simulink model "System_D_passive_simscape"  (R2026a)
settings: Solver=ode23t  StopTime=0.02
libraries: fl_lib x25, nesl_utility x5
settings Model: Creator=mads  LastModifiedBy=mads

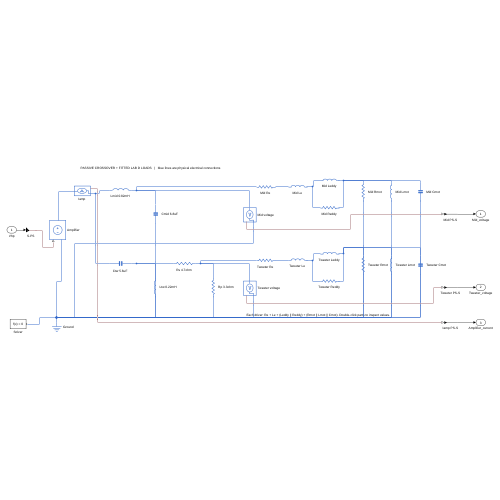
[thumbnail: Simulink's stored preview of the top-level diagram]
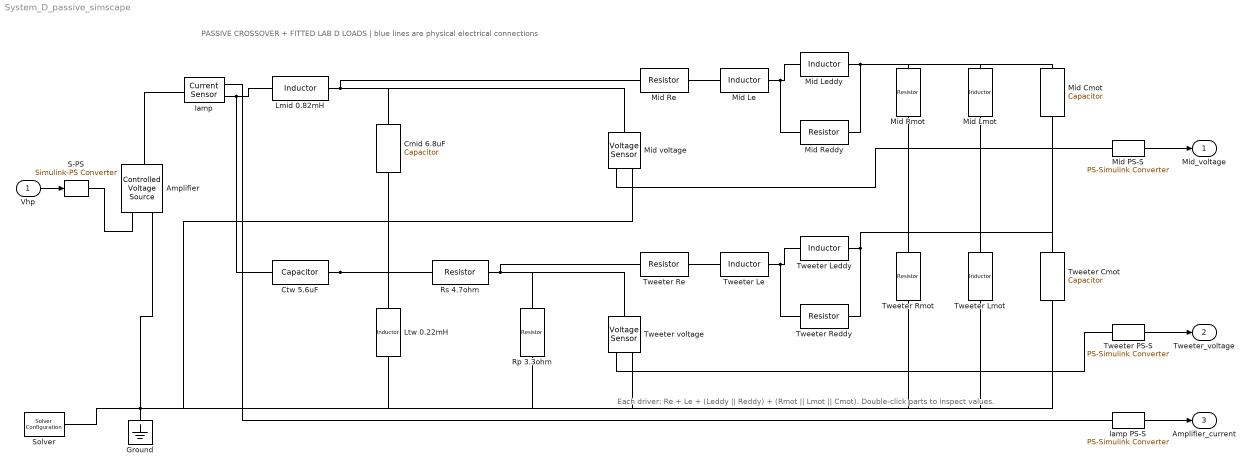
== system System_D_passive_simscape ==
  note: PASSIVE CROSSOVER + FITTED LAB D LOADS | blue lines are physical electrical connections
  note: Each driver: Re + Le + (Leddy || Reddy) + (Rmot || Lmot || Cmot). Double-click parts to inspect values.
  Vhp : Inport
  Amplifier : fl_lib/Electrical/Electrical Sources/Controlled Voltage Source
  Cmid 6.8uF : fl_lib/Electrical/Electrical Elements/Capacitor  c=6.8e-06 F  r=0 Ohm  g=0 1/Ohm  i_specify=off  i_priority=None  i=0 A  i_nominal_specify=off  i_nominal_value=1  i_nominal_unit=A  v_specify=off  v_priority=None  v=0 V  v_nominal_specify=off  v_nominal_value=1  v_nominal_unit=V  vc_specify=off  vc_priority=High  vc=0 V  vc_nominal_specify=off  vc_nominal_value=1  vc_nominal_unit=V
  Ctw 5.6uF : fl_lib/Electrical/Electrical Elements/Capacitor  c=5.6e-06 F  r=0 Ohm  g=0 1/Ohm  i_specify=off  i_priority=None  i=0 A  i_nominal_specify=off  i_nominal_value=1  i_nominal_unit=A  v_specify=off  v_priority=None  v=0 V  v_nominal_specify=off  v_nominal_value=1  v_nominal_unit=V  vc_specify=off  vc_priority=High  vc=0 V  vc_nominal_specify=off  vc_nominal_value=1  vc_nominal_unit=V
  Ground : fl_lib/Electrical/Electrical Elements/Electrical Reference
  Iamp : fl_lib/Electrical/Electrical Sensors/Current Sensor
  Iamp PS-S : nesl_utility/PS-Simulink Converter  PhysicalDomain=network_engine_domain  SubClassName=ps_output  LeftPortType=input  RightPortType=output  PseudoPeriodic=off  Frequencies=[]  VectorFormat=inherit  Unit=A  AffineConversion=off
  Lmid 0.82mH : fl_lib/Electrical/Electrical Elements/Inductor  l=0.00082 H  r=0 Ohm  g=0 1/Ohm  i_specify=off  i_priority=None  i=0 A  i_nominal_specify=off  i_nominal_value=1  i_nominal_unit=A  v_specify=off  v_priority=None  v=0 V  v_nominal_specify=off  v_nominal_value=1  v_nominal_unit=V  i_L_specify=off  i_L_priority=High  i_L=0 A  i_L_nominal_specify=off  i_L_nominal_value=1  i_L_nominal_unit=A
  Ltw 0.22mH : fl_lib/Electrical/Electrical Elements/Inductor  l=0.00022 H  r=0 Ohm  g=0 1/Ohm  i_specify=off  i_priority=None  i=0 A  i_nominal_specify=off  i_nominal_value=1  i_nominal_unit=A  v_specify=off  v_priority=None  v=0 V  v_nominal_specify=off  v_nominal_value=1  v_nominal_unit=V  i_L_specify=off  i_L_priority=High  i_L=0 A  i_L_nominal_specify=off  i_L_nominal_value=1  i_L_nominal_unit=A
  Mid Cmot : fl_lib/Electrical/Electrical Elements/Capacitor  c=0.0004788 F  r=0 Ohm  g=0 1/Ohm  i_specify=off  i_priority=None  i=0 A  i_nominal_specify=off  i_nominal_value=1  i_nominal_unit=A  v_specify=off  v_priority=None  v=0 V  v_nominal_specify=off  v_nominal_value=1  v_nominal_unit=V  vc_specify=off  vc_priority=High  vc=0 V  vc_nominal_specify=off  vc_nominal_value=1  vc_nominal_unit=V
  Mid Le : fl_lib/Electrical/Electrical Elements/Inductor  l=0.0001699 H  r=0 Ohm  g=0 1/Ohm  i_specify=off  i_priority=None  i=0 A  i_nominal_specify=off  i_nominal_value=1  i_nominal_unit=A  v_specify=off  v_priority=None  v=0 V  v_nominal_specify=off  v_nominal_value=1  v_nominal_unit=V  i_L_specify=off  i_L_priority=High  i_L=0 A  i_L_nominal_specify=off  i_L_nominal_value=1  i_L_nominal_unit=A
  Mid Leddy : fl_lib/Electrical/Electrical Elements/Inductor  l=0.0004073 H  r=0 Ohm  g=0 1/Ohm  i_specify=off  i_priority=None  i=0 A  i_nominal_specify=off  i_nominal_value=1  i_nominal_unit=A  v_specify=off  v_priority=None  v=0 V  v_nominal_specify=off  v_nominal_value=1  v_nominal_unit=V  i_L_specify=off  i_L_priority=High  i_L=0 A  i_L_nominal_specify=off  i_L_nominal_value=1  i_L_nominal_unit=A
  Mid Lmot : fl_lib/Electrical/Electrical Elements/Inductor  l=0.006600000000000001 H  r=0 Ohm  g=0 1/Ohm  i_specify=off  i_priority=None  i=0 A  i_nominal_specify=off  i_nominal_value=1  i_nominal_unit=A  v_specify=off  v_priority=None  v=0 V  v_nominal_specify=off  v_nominal_value=1  v_nominal_unit=V  i_L_specify=off  i_L_priority=High  i_L=0 A  i_L_nominal_specify=off  i_L_nominal_value=1  i_L_nominal_unit=A
  Mid PS-S : nesl_utility/PS-Simulink Converter  PhysicalDomain=network_engine_domain  SubClassName=ps_output  LeftPortType=input  RightPortType=output  PseudoPeriodic=off  Frequencies=[]  VectorFormat=inherit  Unit=V  AffineConversion=off
  Mid Re : fl_lib/Electrical/Electrical Elements/Resistor  R=4.6 Ohm  i_specify=off  i_priority=None  i=0 A  i_nominal_specify=off  i_nominal_value=1  i_nominal_unit=A  v_specify=off  v_priority=None  v=0 V  v_nominal_specify=off  v_nominal_value=1  v_nominal_unit=V
  Mid Reddy : fl_lib/Electrical/Electrical Elements/Resistor  R=8.974 Ohm  i_specify=off  i_priority=None  i=0 A  i_nominal_specify=off  i_nominal_value=1  i_nominal_unit=A  v_specify=off  v_priority=None  v=0 V  v_nominal_specify=off  v_nominal_value=1  v_nominal_unit=V
  Mid Rmot : fl_lib/Electrical/Electrical Elements/Resistor  R=14.21262080727686 Ohm  i_specify=off  i_priority=None  i=0 A  i_nominal_specify=off  i_nominal_value=1  i_nominal_unit=A  v_specify=off  v_priority=None  v=0 V  v_nominal_specify=off  v_nominal_value=1  v_nominal_unit=V
  Mid voltage : fl_lib/Electrical/Electrical Sensors/Voltage Sensor
  Rp 3.3ohm : fl_lib/Electrical/Electrical Elements/Resistor  R=3.3 Ohm  i_specify=off  i_priority=None  i=0 A  i_nominal_specify=off  i_nominal_value=1  i_nominal_unit=A  v_specify=off  v_priority=None  v=0 V  v_nominal_specify=off  v_nominal_value=1  v_nominal_unit=V
  Rs 4.7ohm : fl_lib/Electrical/Electrical Elements/Resistor  R=4.7 Ohm  i_specify=off  i_priority=None  i=0 A  i_nominal_specify=off  i_nominal_value=1  i_nominal_unit=A  v_specify=off  v_priority=None  v=0 V  v_nominal_specify=off  v_nominal_value=1  v_nominal_unit=V
  S-PS : nesl_utility/Simulink-PS Converter  PhysicalDomain=network_engine_domain  SubClassName=ps_input  LeftPortType=input  RightPortType=output  PseudoPeriodic=off  Frequencies=[]  NoiseDistribution=none  NoiseParameters=[]  Unit=V  AffineConversion=off  FilteringAndDerivatives=provide  SimscapeFilterOrder=1  InputFilterTimeConstant=0.001  UdotUserProvided=0
  Solver : nesl_utility/Solver Configuration  PhysicalDomain=network_engine_domain  SubClassName=solver  LeftPortType=input  RightPortType=generic  Tones=[]  Harmonics=[]  SimulateNoise=off  Profile=off  UseLocalSampling=off  EnableSwitchedLinearOptims=on  FrequencyDomain=off  UseCCode=off  RelTol=0.001  AbsTol=0.001  MinStep=1e-09  ToWorkspace=off  RevertToSquareIcSolve=off  NumHomotopyIterations=100  PhasorMode=off  PhasorModeNumHarmonics=1  ConsistencySolver=NEWTON_XTOL_AFTER_FTOL  CanonicalOrdering=CANONICAL  OptimizeIntermediates=OPTIMIZED  IndexReductionMethod=DerivativeReplacement  DoDC=off  ResidualTolerance=1e-09  ConsistencyTolSource=GLOBAL  ConsistencyAbsTol=0.001  ConsistencyRelTol=0.001  ConsistencyTolFactor=0.001  UseLocalSolver=off  LocalSolverChoice=NE_BACKWARD_EULER_ADVANCER  ResolveIndetEquations=on  FunctionEvalNumThread=1  LocalSolverSampleTime=0.001  DoFixedCost=off  MaxNonlinIter=3  MaxModeIter=2  ComputeImpulses=off  ImpulseIterations=2  LinearAlgebra=auto  LinearAlgebraNumThread=0  EquationFormulation=NE_TIME_EF  DelaysMemoryBudget=1024  AutomaticFiltering=on  FilteringTimeConstant=0.001  PartitionStorageMethod=AS_NEEDED  PartitionMemoryBudget=1024  PartitionMethod=ROBUST  MultibodyUseLocalSolver=off  MultibodyLocalSolverChoice=ODE1  MultibodyLocalSolverSampleTime=0.001
  Tweeter Cmot : fl_lib/Electrical/Electrical Elements/Capacitor  c=5.582222222222222e-05 F  r=0 Ohm  g=0 1/Ohm  i_specify=off  i_priority=None  i=0 A  i_nominal_specify=off  i_nominal_value=1  i_nominal_unit=A  v_specify=off  v_priority=None  v=0 V  v_nominal_specify=off  v_nominal_value=1  v_nominal_unit=V  vc_specify=off  vc_priority=High  vc=0 V  vc_nominal_specify=off  vc_nominal_value=1  vc_nominal_unit=V
  Tweeter Le : fl_lib/Electrical/Electrical Elements/Inductor  l=1.942e-05 H  r=0 Ohm  g=0 1/Ohm  i_specify=off  i_priority=None  i=0 A  i_nominal_specify=off  i_nominal_value=1  i_nominal_unit=A  v_specify=off  v_priority=None  v=0 V  v_nominal_specify=off  v_nominal_value=1  v_nominal_unit=V  i_L_specify=off  i_L_priority=High  i_L=0 A  i_L_nominal_specify=off  i_L_nominal_value=1  i_L_nominal_unit=A
  Tweeter Leddy : fl_lib/Electrical/Electrical Elements/Inductor  l=2.364e-05 H  r=0 Ohm  g=0 1/Ohm  i_specify=off  i_priority=None  i=0 A  i_nominal_specify=off  i_nominal_value=1  i_nominal_unit=A  v_specify=off  v_priority=None  v=0 V  v_nominal_specify=off  v_nominal_value=1  v_nominal_unit=V  i_L_specify=off  i_L_priority=High  i_L=0 A  i_L_nominal_specify=off  i_L_nominal_value=1  i_L_nominal_unit=A
  Tweeter Lmot : fl_lib/Electrical/Electrical Elements/Inductor  l=0.00022455 H  r=0 Ohm  g=0 1/Ohm  i_specify=off  i_priority=None  i=0 A  i_nominal_specify=off  i_nominal_value=1  i_nominal_unit=A  v_specify=off  v_priority=None  v=0 V  v_nominal_specify=off  v_nominal_value=1  v_nominal_unit=V  i_L_specify=off  i_L_priority=High  i_L=0 A  i_L_nominal_specify=off  i_L_nominal_value=1  i_L_nominal_unit=A
  Tweeter PS-S : nesl_utility/PS-Simulink Converter  PhysicalDomain=network_engine_domain  SubClassName=ps_output  LeftPortType=input  RightPortType=output  PseudoPeriodic=off  Frequencies=[]  VectorFormat=inherit  Unit=V  AffineConversion=off
  Tweeter Re : fl_lib/Electrical/Electrical Elements/Resistor  R=3.4 Ohm  i_specify=off  i_priority=None  i=0 A  i_nominal_specify=off  i_nominal_value=1  i_nominal_unit=A  v_specify=off  v_priority=None  v=0 V  v_nominal_specify=off  v_nominal_value=1  v_nominal_unit=V
  Tweeter Reddy : fl_lib/Electrical/Electrical Elements/Resistor  R=1.577 Ohm  i_specify=off  i_priority=None  i=0 A  i_nominal_specify=off  i_nominal_value=1  i_nominal_unit=A  v_specify=off  v_priority=None  v=0 V  v_nominal_specify=off  v_nominal_value=1  v_nominal_unit=V
  Tweeter Rmot : fl_lib/Electrical/Electrical Elements/Resistor  R=3.106662064204349 Ohm  i_specify=off  i_priority=None  i=0 A  i_nominal_specify=off  i_nominal_value=1  i_nominal_unit=A  v_specify=off  v_priority=None  v=0 V  v_nominal_specify=off  v_nominal_value=1  v_nominal_unit=V
  Tweeter voltage : fl_lib/Electrical/Electrical Sensors/Voltage Sensor
  Mid_voltage : Outport
  Tweeter_voltage : Outport  Port=2
  Amplifier_current : Outport  Port=3
  wires:
  Vhp/1 -> S-PS/1
  Mid PS-S/1 -> Mid_voltage/1
  Tweeter PS-S/1 -> Tweeter_voltage/1
  Iamp PS-S/1 -> Amplifier_current/1
  connections:
  S-PS/RConn1 -- Amplifier/RConn1
  Amplifier/LConn1 -- Iamp/LConn1
  Amplifier/RConn2 -- Solver/RConn1 -- Cmid 6.8uF/RConn1 -- Ltw 0.22mH/RConn1 -- Rp 3.3ohm/RConn1 -- Mid Rmot/RConn1 -- Mid Lmot/RConn1 -- Mid Cmot/RConn1 -- Mid voltage/RConn2 -- Tweeter Rmot/RConn1 -- Tweeter Lmot/RConn1 -- Tweeter Cmot/RConn1 -- Ground/LConn1 -- Tweeter voltage/RConn2
  Lmid 0.82mH/LConn1 -- Iamp/RConn2 -- Ctw 5.6uF/LConn1
  Cmid 6.8uF/LConn1 -- Lmid 0.82mH/RConn1 -- Mid Re/LConn1 -- Mid voltage/LConn1
  Ltw 0.22mH/LConn1 -- Ctw 5.6uF/RConn1 -- Rs 4.7ohm/LConn1
  Rp 3.3ohm/LConn1 -- Rs 4.7ohm/RConn1 -- Tweeter Re/LConn1 -- Tweeter voltage/LConn1
  Mid Re/RConn1 -- Mid Le/LConn1
  Mid Leddy/LConn1 -- Mid Le/RConn1 -- Mid Reddy/LConn1
  Mid Reddy/RConn1 -- Mid Leddy/RConn1 -- Mid Rmot/LConn1 -- Mid Lmot/LConn1 -- Mid Cmot/LConn1
  Mid voltage/RConn1 -- Mid PS-S/LConn1
  Tweeter Re/RConn1 -- Tweeter Le/LConn1
  Tweeter Leddy/LConn1 -- Tweeter Le/RConn1 -- Tweeter Reddy/LConn1
  Tweeter Reddy/RConn1 -- Tweeter Leddy/RConn1 -- Tweeter Rmot/LConn1 -- Tweeter Lmot/LConn1 -- Tweeter Cmot/LConn1
  Tweeter voltage/RConn1 -- Tweeter PS-S/LConn1
  Iamp/RConn1 -- Iamp PS-S/LConn1
